simulink subsystem "rb2_admittance_reference"  (R2024b)
settings: Solver=VariableStepAuto  StartTime=0.0  StopTime=10.0  RelTol=1e-3
undefined symbols (not defined in the file or in its folder): A6, B6
settings Model: Creator=pc  LastModifiedBy=pc

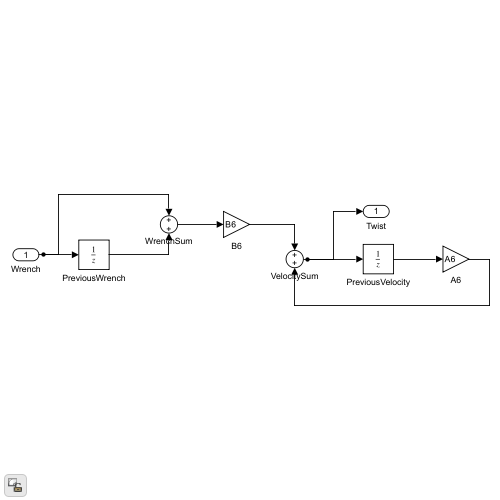
[thumbnail: Simulink's stored preview of the top-level diagram]
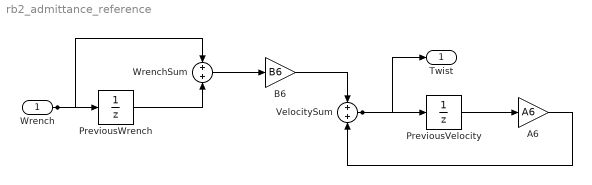
== system rb2_admittance_reference ==
  Wrench : Inport
  A6 : Gain  Gain=A6
  B6 : Gain  Gain=B6
  PreviousVelocity : UnitDelay  InitialCondition=zeros(6,1)  SampleTime=.002  HasFrameUpgradeWarning=on
  PreviousWrench : UnitDelay  InitialCondition=zeros(6,1)  SampleTime=.002  HasFrameUpgradeWarning=on
  VelocitySum : Sum
  WrenchSum : Sum
  Twist : Outport
  wires:
  Wrench/1 -> WrenchSum/1, PreviousWrench/1
  PreviousVelocity/1 -> A6/1
  PreviousWrench/1 -> WrenchSum/2
  A6/1 -> VelocitySum/2
  B6/1 -> VelocitySum/1
  WrenchSum/1 -> B6/1
  VelocitySum/1 -> PreviousVelocity/1, Twist/1
